simulink model "dynamic_function"  (R2023b)
settings: Solver=VariableStepAuto  StartTime=0.0  StopTime=5.5  RelTol=1e-3
undefined symbols (not defined in the file): g, I, L1, L2, M, m, phi
settings Model: Creator=adwei  LastModifiedBy=adwei

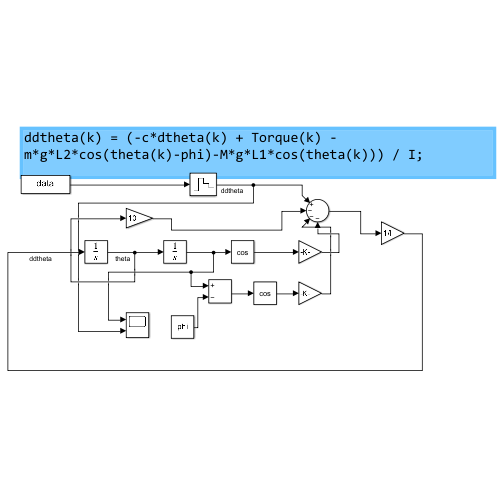
[thumbnail: Simulink's stored preview of the top-level diagram]
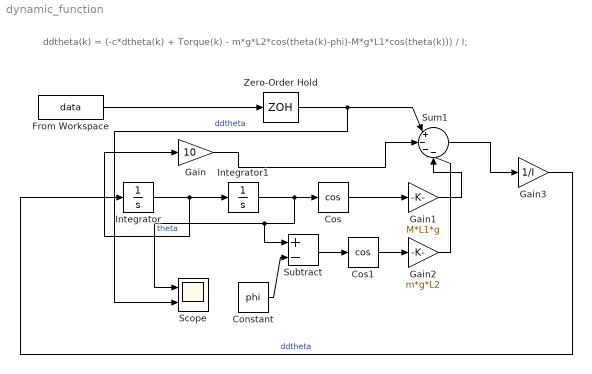
== system dynamic_function ==
  note: ddtheta(k) = (-c*dtheta(k) + Torque(k) - m*g*L2*cos(theta(k)-phi)-M*g*L1*cos(theta(k))) / I;
  Constant : Constant  Value=phi
  Cos : Trigonometry  Operator=cos
  Cos1 : Trigonometry  Operator=cos
  From Workspace : FromWorkspace  VariableName=data
  Gain : Gain  Gain=10
  Gain1 : Gain  Gain=M*L1*g
  Gain2 : Gain  Gain=m*g*L2
  Gain3 : Gain  Gain=1/I
  Integrator : Integrator
  Integrator1 : Integrator  InitialCondition=1.1
  Scope : Scope  NumInputPorts=2
  Subtract : Sum  Inputs=+-
  Sum1 : Sum  Inputs=|+---
  Zero-Order Hold : ZeroOrderHold  SampleTime=0.01
  wires:
  Integrator/1 -> Gain/1, Integrator1/1  "theta"
  Gain/1 -> Sum1/2
  Gain3/1 -> Integrator/1  "ddtheta"
  Cos/1 -> Gain1/1
  Cos1/1 -> Gain2/1
  Subtract/1 -> Cos1/1
  Constant/1 -> Subtract/2
  Zero-Order Hold/1 -> Scope/2, Sum1/1  "ddtheta"
  Gain1/1 -> Sum1/4
  Gain2/1 -> Sum1/3
  Sum1/1 -> Gain3/1
  From Workspace/1 -> Zero-Order Hold/1
  Integrator1/1 -> Scope/1, Subtract/1, Cos/1
